simulink model "MMC_stack_centralized_HAAS_20260927"  (R2024b)
settings: Solver=FixedStepDiscrete  StartTime=t_init_sim  StopTime=sim_time  FixedStep=Ts  RelTol=1e-3
values from neighbouring files (symbols this model uses):
  a = 1    [script_MMC_stack_hackathon_NLM_centralized_HAAS_20260927.m]
  C1low1_active = 1    [script_MMC_stack_hackathon_NLM_centralized_HAAS_20260927.m]
  C2low1_active = 1    [script_MMC_stack_hackathon_NLM_centralized_HAAS_20260927.m]
  C_M_extra = C_m-twist_high_side_C    [script_MMC_stack_hackathon_NLM_centralized_HAAS_20260927.m]
  duty_cycle = 1.0    (= 1)    [script_MMC_stack_hackathon_NLM_centralized_HAAS_20260927.m]
  f0 = 50    [script_MMC_stack_hackathon_NLM_centralized_HAAS_20260927.m]
  feeder_current_lower_rate_limit = -10    [script_MMC_stack_hackathon_NLM_centralized_HAAS_20260927.m]    (also in twist_parameters.m = -500)
  feeder_current_tab = [0.328 0.217 0.162 0.132 0.109 0.094 0.083 0.075 0.068 0.062 0.058 0.054 ... (42 elements, 14x3)]    [feeder_current.mat]
  feeder_current_upper_rate_limit = 0.386/(20e-3)    (= 19.3)    [twist_parameters.m]
  is6VExternallySupplied = true    [script_MMC_stack_hackathon_NLM_centralized_HAAS_20260927.m]
  isFeederJumperOpen = true    [script_MMC_stack_hackathon_NLM_centralized_HAAS_20260927.m]
  L_arm = 30e-3    (= 0.03)    [script_MMC_stack_hackathon_NLM_centralized_HAAS_20260927.m]
  m = 1    [script_MMC_stack_hackathon_NLM_centralized_HAAS_20260927.m]
  N = 5    [script_MMC_stack_hackathon_NLM_centralized_HAAS_20260927.m]
  power_losses = false    [script_MMC_stack_hackathon_NLM_centralized_HAAS_20260927.m]
  R_p = R_s    (= 30)    [script_MMC_stack_hackathon_NLM_centralized_HAAS_20260927.m]
  R_s = 30    [script_MMC_stack_hackathon_NLM_centralized_HAAS_20260927.m]
  source_V = 0    [script_MMC_stack_hackathon_NLM_centralized_HAAS_20260927.m]
  Tcom_sample = round(Tcom / Ts)    [script_MMC_stack_hackathon_NLM_centralized_HAAS_20260927.m]
  time_charge = 0.1    [script_MMC_stack_hackathon_NLM_centralized_HAAS_20260927.m]
  time_decharge = 1.5    [script_MMC_stack_hackathon_NLM_centralized_HAAS_20260927.m]
  Ts = 1e-6    (= 1e-06)    [script_MMC_stack_hackathon_NLM_centralized_HAAS_20260927.m]
  twist_data_acquisition_delay = 50e-9    (= 5e-08)    [script_MMC_stack_hackathon_NLM_centralized_HAAS_20260927.m]    (also in twist_parameters.m)
  twist_data_sampling_period = 1/twist_freq_data_sampling    (= 5e-05)    [script_MMC_stack_hackathon_NLM_centralized_HAAS_20260927.m]    (also in twist_parameters.m)
  twist_dead_time = 200e-9    (= 2e-07)    [twist_parameters.m]
  twist_freq_switching = 200e3    (= 200000)    [twist_parameters.m]
  twist_high_side_adc_R = 1/(1/2e6 + 1/2e6 + 1/(330e3+5.6e3))    (= 251272.836178)    [twist_parameters.m]
  twist_high_side_C = 33e-6*4 + 4.7e-6*12    (= 0.0001884)    [twist_parameters.m]
  twist_high_side_feeder_R = 47e3+4.7e3    (= 51700)    [twist_parameters.m]
  twist_high_side_rC = 0.1    [twist_parameters.m]
  twist_low_side_adc_R = 150e3+470    (= 150470)    [twist_parameters.m]
  twist_low_side_C_ceramic = 3*4.7e-6    (= 1.41e-05)    [twist_parameters.m]
  twist_low_side_C_electrolytic = 47e-6    (= 4.7e-05)    [twist_parameters.m]
  twist_low_side_L = 33e-6    (= 3.3e-05)    [twist_parameters.m]
  twist_low_side_rC = 700e-3    (= 0.7)    [twist_parameters.m]
  twist_low_side_rL = 20e-3    (= 0.02)    [twist_parameters.m]
  twist_R_VCC = (tau_VCC/twist_high_side_C  - twist_high_side_rC)/(1-(tau_VCC/twist_high_side_C - twist_high_side_rC)/R_parallel)    (= 1110.74997822)    [twist_parameters.m]
  VDC = 48    [script_MMC_stack_hackathon_NLM_centralized_HAAS_20260927.m]
undefined symbols (not defined in the file or in its folder): C_SM, feeder_current, gcbh, R, sps_rtmsupport, twist_low_side_lC
libraries: spsSeriesRLCBranchLib x67, spsTriangleGeneratorLib x30, spsMosfetLib x30, spsCurrentMeasurementLib x21, spsVoltageMeasurementLib x17, spsControlledCurrentSourceLib x15, spsDiodeLib x11, spsIdealSwitchLib x10, spsControlledVoltageSourceLib x1, spsGroundLib x1, spspowerguiLib x1
(part 1 of 11)
settings Model: Creator=ana  LastModifiedBy=ana

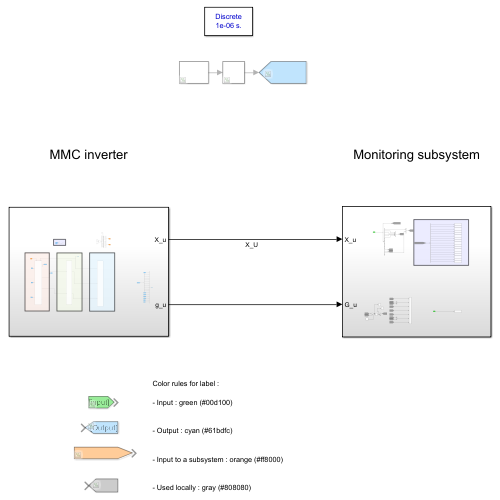
[thumbnail: Simulink's stored preview of the top-level diagram]
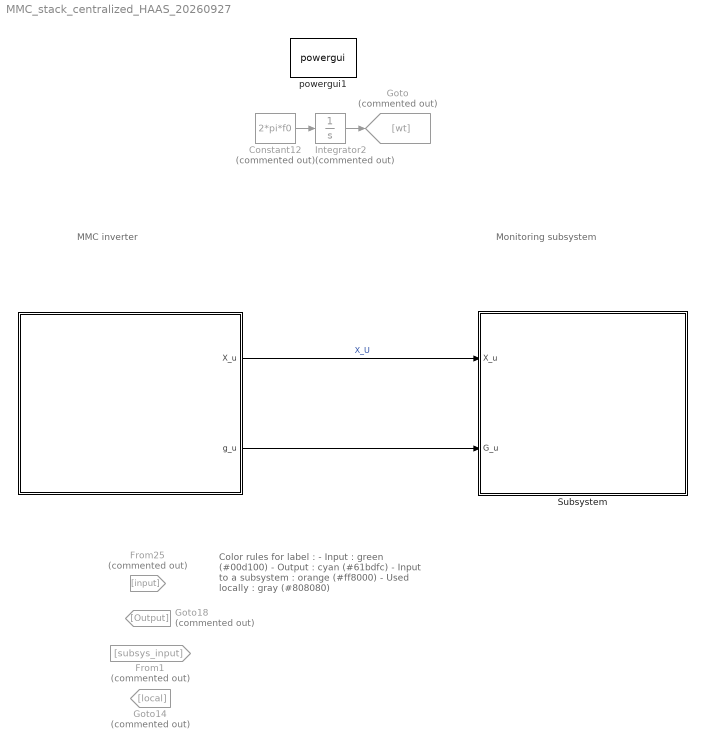
== system MMC_stack_centralized_HAAS_20260927 ==
  note: Color rules for label :
      |
      | - Input : green (#00d100)
      |
      |
      | - Output : cyan (#61bdfc)
      |
      |
      | - Input to a subsystem : orange (#ff8000)
      |
      |
      | - Used locally : gray (#808080)
  note: MMC inverter
  note: Monitoring subsystem
  " " : Subsystem
  Constant12 : Constant  Commented=on  Value=2*pi*f0
  From1 : From  Commented=on  GotoTag=subsys_input
  From25 : From  Commented=on  GotoTag=input
  Goto : Goto  Commented=on  GotoTag=wt
  Goto14 : Goto  Commented=on  GotoTag=local
  Goto18 : Goto  Commented=on  GotoTag=Output
  Integrator2 : Integrator  Commented=on
  Subsystem : Subsystem
  powergui1 : spspowerguiLib/powergui  Priority=1  SimulationMode=Discrete  SampleTime=Ts  frequency=60  Iterations=50  frequencyindice=0  Pbase=100e6  ErrMax=1e-4  UnitsV=V  UnitsW=W  buscounter=0  FunctionMessages=off  echomessages=off  EnableUseOfTLC=off  CurrentSourceSwitches=off  DisableSnubberDevices=off  DisableRonSwitches=off  DisableVfSwitches=off  DisplayEquations=off  AutomaticDiscreteSolvers=off  SolverType=Backward Euler  Interpol=off  ExternalGateDelay=off  methode=off  Ts=0  x0status=blocks  SPID=off  SwTol=0  HookPort=off  NonlinearTolerance=1e-4  nMaxIteration=100  ContinueOnMaxIteration=off  RestoreLinks=warning  ResistiveCurrentMeasurement=off  Frange=[0:2:500]  Ylog=off  Xlog=on  ShowGrid=off  save=off  variable=ZData  structure=0  ZoomFFT=off  StartTime=0.0  cycles=1  DisplayStyle=1  fundamental=60  FreqAxis=off  MaxFrequency=1000  frequencyindicesteady=1  RmsSteady=1  display=off
  wires:
  Constant12/1 -> Integrator2/1
  Integrator2/1 -> Goto/1
  " "/1(X_u) -> Subsystem/1(X_u)  "X_U"
  " "/2(g_u) -> Subsystem/2(G_u)

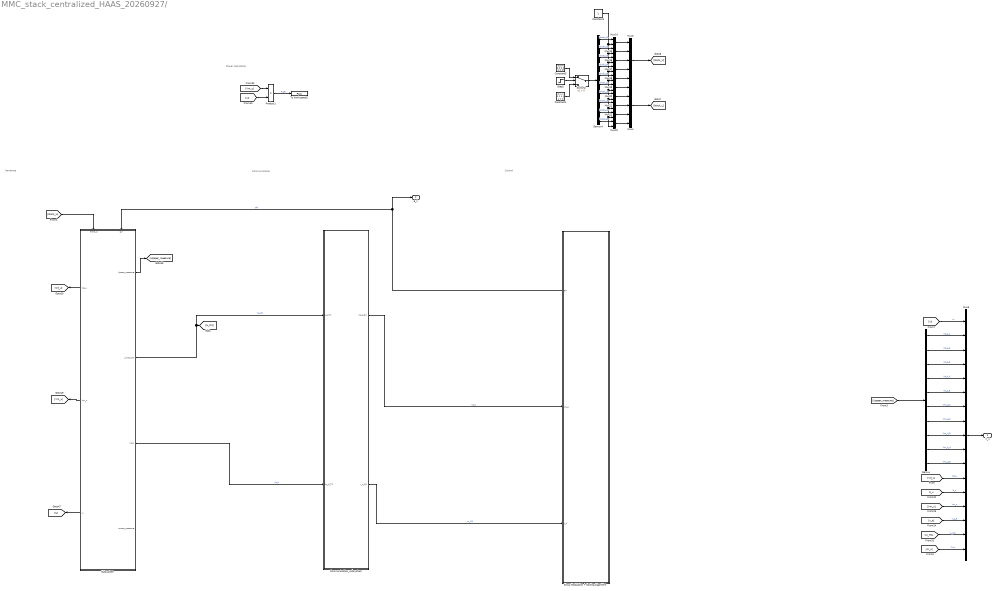
== system MMC_stack_centralized_HAAS_20260927/  ==
  note: Hardware
  note: Communication
  note: Power calculation
  note: Control
  Communication_subsystem : Subsystem
  Constant1 : Constant  Value=[1 1 1 1 1 1 1 1 1 1]
  Constant4 : Constant
  Constant5 : Constant  Value=[0 0 0 0 0 0 0 0 0 0]
  Demux : Demux  Outputs=10
  Demux4 : Demux  Outputs=10
  Mux{14..23} (10 alike) : Mux  Inputs=2
  Mux3 : Mux  Inputs=5
  Mux4 : Mux  Inputs=5
  Mux6 : Mux  Inputs=17
  Product1 : Product
  Sinus Modulation + Sorting Algorithm : Subsystem
      settings: PortSchema="{\"entries\":[{\"content\":{\"sides\":[{\"content\":{\"connectorIds\":[\"Out1\",\"In1\",\"In2\"]},\"type\":\"ConnectorPlacement.EquallySpacedRectSide\",\"uuid\":\"ad0c70b8-bd3d-4dd9-a5c4-c9fd50c7c997\"},{\"content\":{\"side\":\"RIGHT\"},\"type\":\"ConnectorPlacement.EquallySpacedRectSide\",\"uuid\":\"9cc59a2e-07a9-40e0-b04f-27b582e27098\"},{\"content\":{\"side\":\"TOP\"},\"type\":\"ConnectorPlacement.EquallySpacedRectSide\",\"uuid\":\"c85123d6-aff8-40c6-b6df-c7fa366f0af5\"}]},\"type\":\"ConnectorPlacement.EquallySpacedConnector\",\"uuid\":\"b1891b87-83b0-4249-9289-dc35b8395afb\"}],\"packageUris\":[\"http://schema.mathworks.com/mf0/Connector/R2020b\"],\"version\":\"1.0\"}"
  Step2 : Step  Time=time_charge  SampleTime=Ts
  Subsystem : Subsystem
      settings: PortSchema="{\"entries\":[{\"content\":{\"sides\":[{\"content\":{\"connectorIds\":[\"Out5\",\"Out6\",\"Out7\"]},\"type\":\"ConnectorPlacement.EquallySpacedRectSide\",\"uuid\":\"46d0b6b2-241e-4eaa-b5f4-7cb03ad6e4f0\"},{\"content\":{\"connectorIds\":[\"Out1\",\"Out2\",\"Out3\",\"Out4\"],\"side\":\"RIGHT\"},\"type\":\"ConnectorPlacement.EquallySpacedRectSide\",\"uuid\":\"f0391c40-5bbd-42ea-8549-0acba96c1793\"},{\"content\":{\"connectorIds\":[\"In1\",\"In2\"],\"side\":\"TOP\"},\"type\":\"ConnectorPlacement.EquallySpacedRectSide\",\"uuid\":\"1ede63b4-6869-46b3-8b67-84e7db18bcff\"},{\"content\":{\"side\":\"BOTTOM\"},\"type\":\"ConnectorPlacement.EquallySpacedRectSide\",\"uuid\":\"c0e3b199-6126-45b0-9783-8fc4162e2280\"}]},\"type\":\"ConnectorPlacement.EquallySpacedConnector\",\"uuid\":\"8bedc799-aa9e-49e4-9c41-8dbcca404e51\"}],\"packageUris\":[\"http://schema.mathworks.com/mf0/Connector/R2020b\"],\"version\":\"1.0\"}"
  Switch2 : Switch  Criteria=u2 > Threshold  SaturateOnIntegerOverflow=off  InputSameDT=off
  To Workspace2 : ToWorkspace  VariableName=Pout  SaveFormat=Structure With Time  SampleTime=-1
  X_u : Outport
  g_u : Outport  Port=2
  wires:
  Mux6/1 -> X_u/1
  Sinus Modulation + Sorting Algorithm/1(gU) -> Subsystem/2(gU), g_u/1  "gU"
  Communication_subsystem/2(I_U_RX) -> Sinus Modulation + Sorting Algorithm/2(I_U)  "Iu_M1"
  Product1/1 -> To Workspace2/1  "P_sa"
  [iu] -> Product1/2
  [iu] -> Mux6/1  "Iu"
  [Vd_u] -> Mux6/12  "Vd_u"
  [N_u] -> Mux6/13  "N_u"
  [Vm_u] -> Mux6/14  "Vm_u"
  [v_a] -> Mux6/15  "V_s_a"
  [iu_M1] -> Mux6/16  "Iu_M1"
  [Vm_u] -> Product1/1
  Communication_subsystem/1(Vc_U_RX) -> Sinus Modulation + Sorting Algorithm/1(Vc_U)  "Vc_U"
  [Uppper_measure] -> Demux/1
  Demux/1 -> Mux6/2  "Vc_U_1"
  Demux/2 -> Mux6/3  "Vc_U_2"
  Demux/3 -> Mux6/4  "Vc_U_3"
  Demux/4 -> Mux6/5  "Vc_U_4"
  Demux/5 -> Mux6/6  "Vc_U_5"
  Demux/6 -> Mux6/7  "Vm_U_1"
  Demux/7 -> Mux6/8  "Vm_U_2"
  Demux/8 -> Mux6/9  "Vm_U_3"
  Demux/9 -> Mux6/10  "Vm_U_4"
  Demux/10 -> Mux6/11  "Vm_U_5"
  [m_u] -> Mux6/17  "m_u"
  Subsystem/2(i_mod_M1) -> Communication_subsystem/1(I_U_TX), [iu_M1]  "IU_M1"
  Subsystem/3(Vc_U) -> Communication_subsystem/2(Vc_U_TX)  "Vc_U"
  Subsystem/7(iu) -> [iu]
  Subsystem/6(Vm_u) -> [Vm_u]
  Subsystem/5(Vd_u) -> [Vd_u]
  Subsystem/1(Upper_measure) -> [Uppper_measure]
  [block_U] -> Subsystem/1(block_U)
  Demux4/9 -> Mux22/1  "block_L4"
  Mux17/1 -> Mux3/4
  Mux22/1 -> Mux4/4
  Mux14/1 -> Mux3/1
  Demux4/1 -> Mux14/1  "block_U1"
  Constant5/1 -> Switch2/1
  Demux4/3 -> Mux16/1  "block_U3"
  Mux21/1 -> Mux4/3
  Switch2/1 -> Demux4/1
  Demux4/5 -> Mux18/1  "block_U5"
  Demux4/10 -> Mux23/1  "block_L5"
  Constant1/1 -> Switch2/3
  Demux4/7 -> Mux20/1  "block_L2"
  Mux19/1 -> Mux4/1
  Mux23/1 -> Mux4/5
  Demux4/2 -> Mux15/1  "block_U2"
  Constant4/1 -> Mux23/2, Mux22/2, Mux21/2, Mux20/2, Mux19/2, Mux18/2, Mux17/2, Mux16/2, Mux15/2, Mux14/2
  Demux4/6 -> Mux19/1  "block_L1"
  Demux4/8 -> Mux21/1  "block_L3"
  Mux16/1 -> Mux3/3
  Mux15/1 -> Mux3/2
  Mux20/1 -> Mux4/2
  Mux18/1 -> Mux3/5
  Demux4/4 -> Mux17/1  "block_U4"
  Step2/1 -> Switch2/2
  Mux3/1 -> [block_U]
  Mux4/1 -> [block_L]

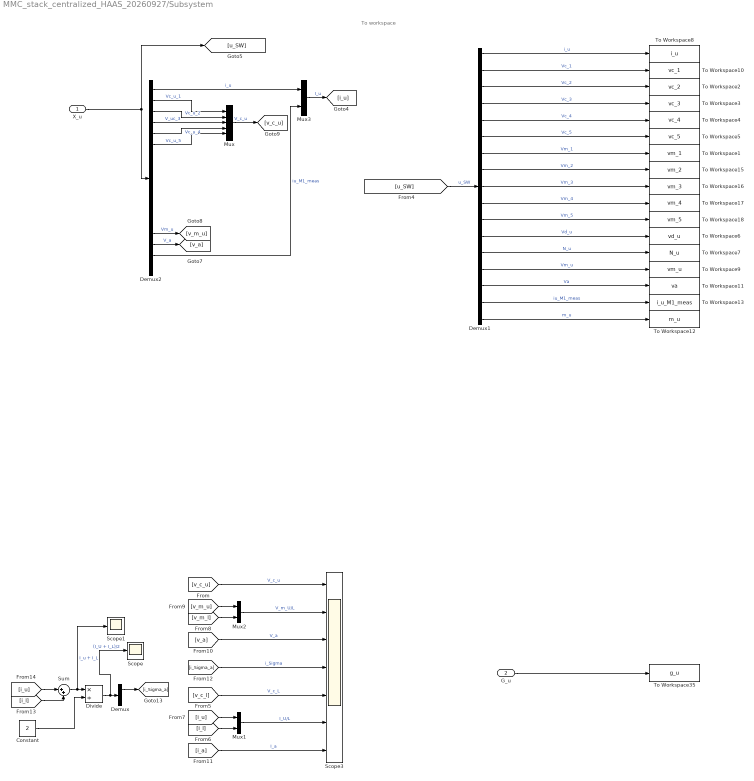
== system MMC_stack_centralized_HAAS_20260927/Subsystem ==
  note: To workspace
  X_u : Inport
  G_u : Inport  Port=2
  Constant : Constant  Value=2
  Demux : Demux  Outputs=2
  Demux1 : Demux  Outputs=17
  Demux2 : Demux  Outputs=17
  Divide : Product  Inputs=*/
  Mux : Mux  Inputs=5
  Mux1 : Mux  Inputs=2
  Mux2 : Mux  Inputs=2
  Mux3 : Mux  Inputs=2
  Scope : Scope
  Scope1 : Scope
  Scope3 : Scope  NumInputPorts=7
  Sum : Sum  Inputs=|++
  To Workspace1 : ToWorkspace  VariableName=vm_1  SaveFormat=Structure With Time  SampleTime=-1
  To Workspace10 : ToWorkspace  VariableName=vc_1  SaveFormat=Structure With Time  SampleTime=-1
  To Workspace11 : ToWorkspace  VariableName=va  SaveFormat=Structure With Time  SampleTime=-1
  To Workspace12 : ToWorkspace  VariableName=m_u  SaveFormat=Structure With Time  SampleTime=-1
  To Workspace13 : ToWorkspace  VariableName=i_u_M1_meas  SaveFormat=Structure With Time  SampleTime=-1
  To Workspace15 : ToWorkspace  VariableName=vm_2  SaveFormat=Structure With Time  SampleTime=-1
  To Workspace16 : ToWorkspace  VariableName=vm_3  SaveFormat=Structure With Time  SampleTime=-1
  To Workspace17 : ToWorkspace  VariableName=vm_4  SaveFormat=Structure With Time  SampleTime=-1
  To Workspace18 : ToWorkspace  VariableName=vm_5  SaveFormat=Structure With Time  SampleTime=-1
  To Workspace2 : ToWorkspace  VariableName=vc_2  SaveFormat=Structure With Time  SampleTime=-1
  To Workspace3 : ToWorkspace  VariableName=vc_3  SaveFormat=Structure With Time  SampleTime=-1
  To Workspace35 : ToWorkspace  VariableName=g_u  SaveFormat=Structure With Time  SampleTime=-1
  To Workspace4 : ToWorkspace  VariableName=vc_4  SaveFormat=Structure With Time  SampleTime=-1
  To Workspace5 : ToWorkspace  VariableName=vc_5  SaveFormat=Structure With Time  SampleTime=-1
  To Workspace6 : ToWorkspace  VariableName=vd_u  SaveFormat=Structure With Time  SampleTime=-1
  To Workspace7 : ToWorkspace  VariableName=N_u  SaveFormat=Structure With Time  SampleTime=-1
  To Workspace8 : ToWorkspace  VariableName=i_u  SaveFormat=Structure With Time  SampleTime=-1
  To Workspace9 : ToWorkspace  VariableName=vm_u  SaveFormat=Structure With Time  SampleTime=-1
  wires:
  Demux1/4 -> To Workspace3/1  "Vc_3"
  Demux2/14 -> [v_m_u]  "Vm_u"
  Demux1/2 -> To Workspace10/1  "Vc_1"
  Demux1/14 -> To Workspace9/1  "Vm_u"
  Mux2/1 -> Scope3/2  "V_m_U/L"
  Demux1/7 -> To Workspace1/1  "Vm_1"
  Demux2/1 -> Mux3/1  "i_u"
  Demux2/4 -> Mux/3  "V_uc_3"
  [v_m_u] -> Mux2/1
  [i_a] -> Scope3/7  "I_a"
  X_u/1 -> Demux2/1, [u_SW]
  Demux2/15 -> [v_a]  "V_a"
  Demux2/16 -> Mux3/2  "iu_M1_meas"
  [i_l] -> Sum/2
  Demux1/11 -> To Workspace18/1  "Vm_5"
  Demux1/13 -> To Workspace7/1  "N_u"
  Demux2/3 -> Mux/2  "Vc_u_2"
  [i_u] -> Mux1/1
  Demux1/5 -> To Workspace4/1  "Vc_4"
  Mux3/1 -> [i_u]  "I_u"
  Constant/1 -> Divide/2
  Sum/1 -> Scope1/1, Divide/1  "I_u + I_L"
  Divide/1 -> Scope/1, Demux/1  "(I_U + I_L)/2"
  Demux1/3 -> To Workspace2/1  "Vc_2"
  Demux1/16 -> To Workspace13/1  "iu_M1_meas"
  Demux2/5 -> Mux/4  "Vc_u_4"
  [v_a] -> Scope3/3  "V_a"
  Demux1/10 -> To Workspace17/1  "Vm_4"
  [i_l] -> Mux1/2
  [u_SW] -> Demux1/1  "u_SW"
  Demux1/17 -> To Workspace12/1  "m_u"
  Demux1/15 -> To Workspace11/1  "Va"
  Demux1/12 -> To Workspace6/1  "Vd_u"
  Demux2/2 -> Mux/1  "Vc_u_1"
  Demux1/9 -> To Workspace16/1  "Vm_3"
  Demux/1 -> [i_Sigma_a]
  [v_c_l] -> Scope3/5  "V_c_L"
  Demux2/6 -> Mux/5  "Vc_u_5"
  Demux1/8 -> To Workspace15/1  "Vm_2"
  [v_c_u] -> Scope3/1  "V_c_u"
  Demux1/6 -> To Workspace5/1  "Vc_5"
  Demux1/1 -> To Workspace8/1  "i_u"
  [v_m_l] -> Mux2/2
  [i_u] -> Sum/1
  [i_Sigma_a] -> Scope3/4  "i_Sigma"
  Mux1/1 -> Scope3/6  "I_U/L"
  Mux/1 -> [v_c_u]  "V_c_u"
  G_u/1 -> To Workspace35/1

== system MMC_stack_centralized_HAAS_20260927/ /Communication_subsystem ==
  I_U_TX : Inport
  Vc_U_TX : Inport  Port=2
  Communication architecture : Subsystem
      settings: PortSchema="{\"entries\":[{\"content\":{\"sides\":[{\"content\":{\"connectorIds\":[\"In1\",\"In2\",\"Out2\",\"In3\",\"Out3\",\"In4\",\"Out4\",\"In5\",\"Out5\",\"Out6\"]},\"type\":\"ConnectorPlacement.EquallySpacedRectSide\",\"uuid\":\"574f1c32-5c90-4713-aad2-348eca17c1e3\"},{\"content\":{\"connectorIds\":[\"Out1\"],\"side\":\"RIGHT\"},\"type\":\"ConnectorPlacement.EquallySpacedRectSide\",\"uuid\":\"f8c779b5-ecb7-4a42-bc9c-e4bb2f97a0b3\"},{\"content\":{\"side\":\"TOP\"},\"type\":\"ConnectorPlacement.EquallySpacedRectSide\",\"uuid\":\"aac8d141-a504-4135-a079-04baa73dba14\"}]},\"type\":\"ConnectorPlacement.EquallySpacedConnector\",\"uuid\":\"cbc34fff-d47b-42f9-bfde-18f06952df39\"}],\"packageUris\":[\"http://schema.mathworks.com/mf0/Connector/R2020b\"],\"version\":\"1.0\"}"
  Demux2 : Demux  Outputs=12
  Mux : Mux  Inputs=2
  Scope : Scope
  Sync : DiscretePulseGenerator  Period=round((200e-6)/Ts)  PulseWidth=round(20e-6/Ts)  SampleTime=Ts
  Term_RX_{7..12} (6 alike) : Terminator
  Upper_arm : Subsystem
      settings: PortSchema="{\"entries\":[{\"content\":{\"sides\":[{\"content\":{\"connectorIds\":[\"In1\",\"In2\"]},\"type\":\"ConnectorPlacement.EquallySpacedRectSide\",\"uuid\":\"e2448297-5920-4ed4-b9a5-463387ed0389\"},{\"content\":{\"connectorIds\":[\"Out1\",\"In3\",\"Out2\",\"In4\",\"Out3\",\"In5\",\"Out4\",\"In6\",\"Out5\",\"In7\"],\"side\":\"RIGHT\"},\"type\":\"ConnectorPlacement.EquallySpacedRectSide\",\"uuid\":\"29ac6558-0bf6-4432-86a8-2cc792ef1820\"},{\"content\":{\"connectorIds\":[\"Out6\"],\"side\":\"TOP\"},\"type\":\"ConnectorPlacement.EquallySpacedRectSide\",\"uuid\":\"fe3a666d-35d9-4a5d-8998-edcd1cd24e1f\"}]},\"type\":\"ConnectorPlacement.EquallySpacedConnector\",\"uuid\":\"a9564cd0-ea30-4b39-994d-f524846fcfc7\"}],\"packageUris\":[\"http://schema.mathworks.com/mf0/Connector/R2020b\"],\"version\":\"1.0\"}"
  Vector Concatenate : Concatenate  NumInputs=5
  Vc_U_RX : Outport
  I_U_RX : Outport  Port=2
  wires:
  Vc_U_TX/1 -> Mux/1
  Mux/1 -> Upper_arm/1(upper_arm_info)
  Upper_arm/1(M1_TX_signal) -> Communication architecture/1(M1_TX_Signal)
  Upper_arm/2(M2_TX_signal) -> Communication architecture/2(M2_TX_Signal)
  Upper_arm/3(M3_TX_signal) -> Communication architecture/3(M3_TX_Signal)
  Upper_arm/4(M4_TX_signal) -> Communication architecture/4(M4_TX_Signal)
  Upper_arm/5(M5_TX_signal) -> Communication architecture/5(M5_TX_Signal)
  I_U_TX/1 -> Mux/2
  Sync/1 -> Upper_arm/2(sync)
  Upper_arm/6(RX_Variables) -> [RX_variable]
  [RX_variable] -> Demux2/1
  Demux2/1 -> Scope/1, Vector Concatenate/1  "Vc_u_1"
  Demux2/2 -> Vector Concatenate/2  "Vc_u_2"
  Demux2/3 -> Vector Concatenate/3  "Vc_u_3"
  Demux2/4 -> Vector Concatenate/4  "Vc_u_4"
  Demux2/5 -> Vector Concatenate/5  "Vc_u_5"
  Vector Concatenate/1 -> Vc_U_RX/1
  Demux2/6 -> I_U_RX/1
  Communication architecture/2(M2_RX_Signal) -> Upper_arm/4(M2_RX_signal)
  Communication architecture/3(M3_RX_Signal) -> Upper_arm/5(M3_RX_signal)
  Communication architecture/4(M4_RX_Signal) -> Upper_arm/6(M4_RX_signal)
  Communication architecture/5(M5_RX_Signal) -> Upper_arm/7(M5_RX_signal)
  Communication architecture/6(M1_RX_Signal) -> Upper_arm/3(M1_RX_signal)
  Demux2/7 -> Term_RX_7/1
  Demux2/8 -> Term_RX_8/1
  Demux2/9 -> Term_RX_9/1
  Demux2/10 -> Term_RX_10/1
  Demux2/11 -> Term_RX_11/1
  Demux2/12 -> Term_RX_12/1

== system MMC_stack_centralized_HAAS_20260927/ /Sinus Modulation + Sorting Algorithm ==
  note: Sorting and CVB algorithm - Upper and Lower stacks
  note: Gate assignement - Modules MCUs
  Vc_U : Inport
  I_U : Inport  Port=2
  Constant5 : Constant
  Constant6 : Constant  Value=2
  Constant7 : Constant  Value=3
  Constant8 : Constant  Value=4
  Constant9 : Constant  Value=5
  M1 MCU : Subsystem
  M2 MCU : Subsystem
  M3 MCU : Subsystem
  M4 MCU : Subsystem
  M5 MCU : Subsystem
  Mux : Mux  Inputs=5
  Supervisor MCU : Subsystem
  gU : Outport
  tag scope: g_u_supervisor=global
  wires:
  M1 MCU/1(g_unitaire_stack) -> Mux/1
  M2 MCU/1(g_unitaire_stack) -> Mux/2
  M3 MCU/1(g_unitaire_stack) -> Mux/3
  M4 MCU/1(g_unitaire_stack) -> Mux/4
  M5 MCU/1(g_unitaire_stack) -> Mux/5
  Constant5/1 -> M1 MCU/2(M_number)
  Constant6/1 -> M2 MCU/2(M_number)
  Constant7/1 -> M3 MCU/2(M_number)
  Constant8/1 -> M4 MCU/2(M_number)
  Constant9/1 -> M5 MCU/2(M_number)
  I_U/1 -> Supervisor MCU/2(I_U)
  Vc_U/1 -> Supervisor MCU/1(Vc_U)
  Supervisor MCU/1(gU) -> [g_u_supervisor]
  [g_u_supervisor] -> M5 MCU/1(g_u), M4 MCU/1(g_u), M3 MCU/1(g_u), M2 MCU/1(g_u), M1 MCU/1(g_u)
  Mux/1 -> gU/1

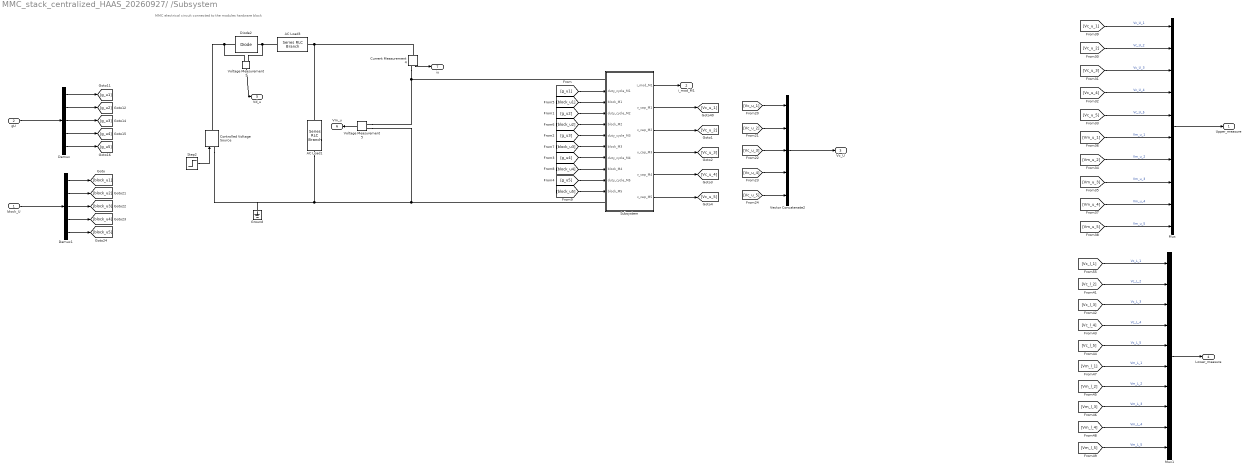
== system MMC_stack_centralized_HAAS_20260927/ /Subsystem ==
  note: MMC electrical circuit connected to the modules hardware block
  block_U : Inport
  gU : Inport  Port=2
  AC Load1 : spsSeriesRLCBranchLib/Series RLC Branch  LConnTagsString=__new0  RConnTagsString=__new0  BranchType=R  Resistance=R_p  Inductance=L_arm  SetiL0=off  InitialCurrent=0  Capacitance=C_SM  Setx0=off  InitialVoltage=0  Measurements=None
  AC Load3 : spsSeriesRLCBranchLib/Series RLC Branch  LConnTagsString=__new0  RConnTagsString=__new0  BranchType=R  Resistance=R_s  Inductance=L_arm  SetiL0=off  InitialCurrent=0  Capacitance=C_SM  Setx0=off  InitialVoltage=0  Measurements=None
  Controlled Voltage Source : spsControlledVoltageSourceLib/Controlled Voltage Source  Initialize=on  Source_Type=DC  Amplitude=0  Phase=0  Frequency=0  Measurements=None
  Current Measurement4 : spsCurrentMeasurementLib/Current Measurement  PhasorSimulation=off  OutputType=Complex  PSBequivalent=0
  Demux : Demux  Outputs=5
  Demux1 : Demux  Outputs=5
  Diode2 : spsDiodeLib/Diode  Ron=0.001  Lon=0  Vf=0.8  IC=0  UseSnubber=0  Rs=1e5  Cs=inf  Measurements=off
  Ground : spsGroundLib/Ground  LConnTagsString=a
  Mux : Mux  Inputs=10
  Mux1 : Mux  Inputs=10
  Step2 : Step  Time=time_decharge  Before=VDC  After=0  SampleTime=0
  Subsystem : Subsystem
      settings: PortSchema="{\"entries\":[{\"content\":{\"sides\":[{\"content\":{\"connectorIds\":[\"LConn1\",\"In1\",\"In2\",\"In3\",\"In4\",\"In5\",\"In6\",\"In7\",\"In8\",\"In9\",\"In10\",\"LConn2\"]},\"type\":\"ConnectorPlacement.EquallySpacedRectSide\",\"uuid\":\"af96ca56-9fdb-47ea-8e31-50f481daafc4\"},{\"content\":{\"connectorIds\":[\"Out1\",\"Out2\",\"Out3\",\"Out4\",\"Out5\",\"Out6\"],\"side\":\"RIGHT\"},\"type\":\"ConnectorPlacement.EquallySpacedRectSide\",\"uuid\":\"66f6256f-049a-4c8a-aad5-8d93b148b037\"},{\"content\":{\"side\":\"TOP\"},\"type\":\"ConnectorPlacement.EquallySpacedRectSide\",\"uuid\":\"596eb3e1-7761-4783-802e-d9df31b3a9c1\"}]},\"type\":\"ConnectorPlacement.EquallySpacedConnector\",\"uuid\":\"34c6ade5-a2f4-48d8-9a9b-6856a5a88d76\"}],\"packageUris\":[\"http://schema.mathworks.com/mf0/Connector/R2020b\"],\"version\":\"1.0\"}"
  Vector Concatenate2 : Concatenate  NumInputs=5
  Voltage Measurement5 : spsVoltageMeasurementLib/Voltage Measurement  PhasorSimulation=off  OutputType=Complex  PSBequivalent=0
  Voltage Measurement7 : spsVoltageMeasurementLib/Voltage Measurement  PhasorSimulation=off  OutputType=Complex  PSBequivalent=0
  Upper_measure : Outport
  i_mod_M1 : Outport  Port=2
  Vc_U : Outport  Port=3
  Lower_measure : Outport  Port=4
  Vd_u : Outport  Port=5
  Vm_u : Outport  Port=6
  iu : Outport  Port=7
  wires:
  Voltage Measurement7/1 -> Vd_u/1
  Step2/1 -> Controlled Voltage Source/1
  Voltage Measurement5/1 -> Vm_u/1
  [g_u1] -> Subsystem/1(duty_cycle_M1)
  [block_u1] -> Subsystem/2(block_M1)
  [g_u2] -> Subsystem/3(duty_cycle_M2)
  [block_u2] -> Subsystem/4(block_M2)
  [g_u3] -> Subsystem/5(duty_cycle_M3)
  [block_u3] -> Subsystem/6(block_M3)
  [g_u4] -> Subsystem/7(duty_cycle_M4)
  [block_u4] -> Subsystem/8(block_M4)
  [g_u5] -> Subsystem/9(duty_cycle_M5)
  [block_u5] -> Subsystem/10(block_M5)
  Subsystem/1(i_mod_M1) -> i_mod_M1/1
  Subsystem/6(v_cap_M5) -> [Vc_u_5]
  Subsystem/5(v_cap_M4) -> [Vc_u_4]
  Subsystem/2(v_cap_M1) -> [Vc_u_1]
  Subsystem/3(v_cap_M2) -> [Vc_u_2]
  Subsystem/4(v_cap_M3) -> [Vc_u_3]
  Current Measurement4/1 -> iu/1
  Vector Concatenate2/1 -> Vc_U/1
  Demux/2 -> [g_u2]
  Demux/5 -> [g_u5]
  Demux1/5 -> [block_u5]
  Demux/4 -> [g_u4]
  Demux/3 -> [g_u3]
  Demux1/1 -> [block_u1]
  gU/1 -> Demux/1
  block_U/1 -> Demux1/1
  Demux1/2 -> [block_u2]
  Demux/1 -> [g_u1]
  Demux1/4 -> [block_u4]
  Demux1/3 -> [block_u3]
  [Vc_u_1] -> Vector Concatenate2/1
  [Vc_u_2] -> Vector Concatenate2/2
  [Vc_u_3] -> Vector Concatenate2/3
  [Vc_u_4] -> Vector Concatenate2/4
  [Vc_u_5] -> Vector Concatenate2/5
  [Vc_u_1] -> Mux/1  "Vc_U_1"
  [Vm_u_5] -> Mux/10  "Vm_u_5"
  [Vm_u_4] -> Mux/9  "Vm_u_4"
  [Vc_u_3] -> Mux/3  "Vc_U_3"
  [Vm_u_3] -> Mux/8  "Vm_u_3"
  [Vc_u_2] -> Mux/2  "Vc_U_2"
  [Vm_u_2] -> Mux/7  "Vm_u_2"
  [Vm_u_1] -> Mux/6  "Vm_u_1"
  [Vc_u_4] -> Mux/4  "Vc_U_4"
  [Vc_u_5] -> Mux/5  "Vc_U_5"
  [Vc_l_2] -> Mux1/2  "Vc_L_2"
  [Vm_l_2] -> Mux1/7  "Vm_L_2"
  [Vc_l_1] -> Mux1/1  "Vc_L_1"
  [Vm_l_4] -> Mux1/9  "Vm_L_4"
  [Vm_l_5] -> Mux1/10  "Vm_L_5"
  [Vm_l_1] -> Mux1/6  "Vm_L_1"
  [Vm_l_3] -> Mux1/8  "Vm_L_3"
  [Vc_l_3] -> Mux1/3  "Vc_L_3"
  [Vc_l_5] -> Mux1/5  "Vc_L_5"
  [Vc_l_4] -> Mux1/4  "Vc_L_4"
  Mux1/1 -> Lower_measure/1
  Mux/1 -> Upper_measure/1
  connections:
  Diode2/RConn1 -- AC Load3/LConn1 -- Voltage Measurement7/LConn2
  Current Measurement4/RConn1 -- Voltage Measurement5/LConn1 -- Subsystem/LConn1
  Voltage Measurement5/LConn2 -- Controlled Voltage Source/LConn1 -- Ground/LConn1 -- AC Load1/RConn1 -- Subsystem/LConn2
  Voltage Measurement7/LConn1 -- Controlled Voltage Source/RConn1 -- Diode2/LConn1
  AC Load1/LConn1 -- Current Measurement4/LConn1 -- AC Load3/RConn1

== system MMC_stack_centralized_HAAS_20260927/ /Communication_subsystem/Communication architecture ==
  M1_TX_Signal : Inport
  M2_TX_Signal : Inport  Port=2
  M3_TX_Signal : Inport  Port=3
  M4_TX_Signal : Inport  Port=4
  M5_TX_Signal : Inport  Port=5
  MATLAB Function : MATLAB Function  Commented=on  TreatAsAtomicUnit=on
  RX_Signal : Outport
  M2_RX_Signal : Outport  Port=2
  M3_RX_Signal : Outport  Port=3
  M4_RX_Signal : Outport  Port=4
  M5_RX_Signal : Outport  Port=5
  M1_RX_Signal : Outport  Port=6
  wires:
  MATLAB Function/1(bus_signal) -> RX_Signal/1
  M4_TX_Signal/1 -> M5_RX_Signal/1
  M5_TX_Signal/1 -> M1_RX_Signal/1
  M1_TX_Signal/1 -> M2_RX_Signal/1
  M2_TX_Signal/1 -> M3_RX_Signal/1
  M3_TX_Signal/1 -> M4_RX_Signal/1

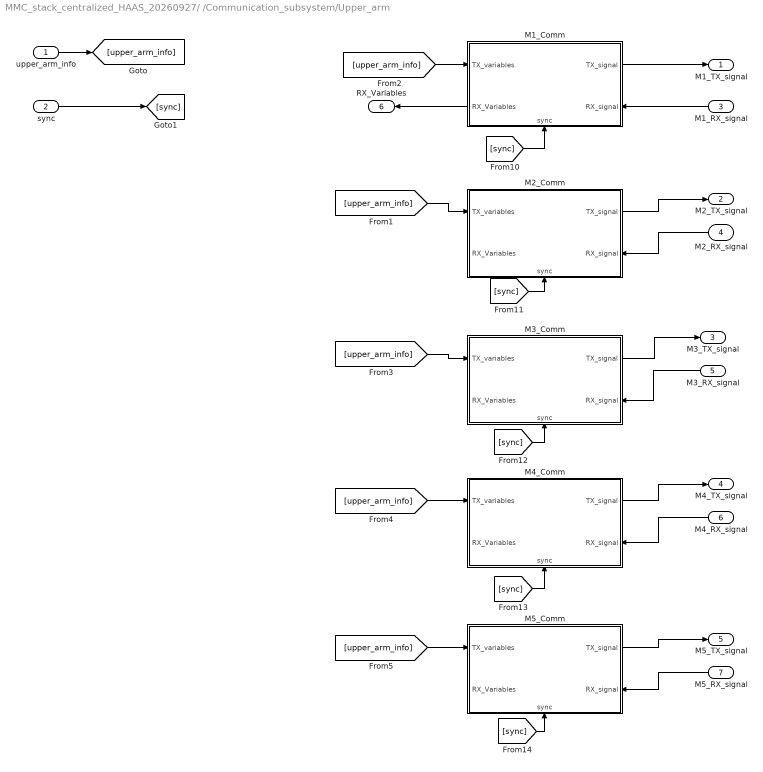
== system MMC_stack_centralized_HAAS_20260927/ /Communication_subsystem/Upper_arm ==
  upper_arm_info : Inport
  sync : Inport  Port=2
  M1_RX_signal : Inport  Port=3
  M2_RX_signal : Inport  Port=4
  M3_RX_signal : Inport  Port=5
  M4_RX_signal : Inport  Port=6
  M5_RX_signal : Inport  Port=7
  M1_Comm : Subsystem
      settings: PortSchema="{\"entries\":[{\"content\":{\"sides\":[{\"content\":{\"connectorIds\":[\"In1\",\"Out2\"]},\"type\":\"ConnectorPlacement.EquallySpacedRectSide\",\"uuid\":\"c3733cfa-9814-4ae5-a55a-8e5b6f8a57d7\"},{\"content\":{\"connectorIds\":[\"Out1\",\"In3\"],\"side\":\"RIGHT\"},\"type\":\"ConnectorPlacement.EquallySpacedRectSide\",\"uuid\":\"d16535d3-81ee-4162-a646-15cef1f1639a\"},{\"content\":{\"side\":\"TOP\"},\"type\":\"ConnectorPlacement.EquallySpacedRectSide\",\"uuid\":\"672d53ef-99b6-4fa6-8351-42251f607454\"},{\"content\":{\"connectorIds\":[\"In2\"],\"side\":\"BOTTOM\"},\"type\":\"ConnectorPlacement.EquallySpacedRectSide\",\"uuid\":\"a9bd7512-44c2-4af9-8132-4c17be33b3c2\"}]},\"type\":\"ConnectorPlacement.EquallySpacedConnector\",\"uuid\":\"554aea8b-7fd0-4035-ac75-3acab423d605\"}],\"packageUris\":[\"http://schema.mathworks.com/mf0/Connector/R2020b\"],\"version\":\"1.0\"}"
  M2_Comm : Subsystem
      settings: PortSchema="{\"entries\":[{\"content\":{\"sides\":[{\"content\":{\"connectorIds\":[\"In1\",\"Out2\"]},\"type\":\"ConnectorPlacement.EquallySpacedRectSide\",\"uuid\":\"47077a1e-eba1-4129-8203-93262b2de465\"},{\"content\":{\"connectorIds\":[\"Out1\",\"In3\"],\"side\":\"RIGHT\"},\"type\":\"ConnectorPlacement.EquallySpacedRectSide\",\"uuid\":\"701fdbad-c928-45f3-8ba2-a14f680316f8\"},{\"content\":{\"side\":\"TOP\"},\"type\":\"ConnectorPlacement.EquallySpacedRectSide\",\"uuid\":\"d648951b-caea-4569-a411-8455254fdbc0\"},{\"content\":{\"connectorIds\":[\"In2\"],\"side\":\"BOTTOM\"},\"type\":\"ConnectorPlacement.EquallySpacedRectSide\",\"uuid\":\"d4b1d2d6-b4a1-4e2c-9ca6-248db102ef7c\"}]},\"type\":\"ConnectorPlacement.EquallySpacedConnector\",\"uuid\":\"7c33ff72-602e-419f-9c2d-5eefc0d60400\"}],\"packageUris\":[\"http://schema.mathworks.com/mf0/Connector/R2020b\"],\"version\":\"1.0\"}"
  M3_Comm : Subsystem
      settings: PortSchema="{\"entries\":[{\"content\":{\"sides\":[{\"content\":{\"connectorIds\":[\"In1\",\"Out2\"]},\"type\":\"ConnectorPlacement.EquallySpacedRectSide\",\"uuid\":\"47077a1e-eba1-4129-8203-93262b2de465\"},{\"content\":{\"connectorIds\":[\"Out1\",\"In3\"],\"side\":\"RIGHT\"},\"type\":\"ConnectorPlacement.EquallySpacedRectSide\",\"uuid\":\"701fdbad-c928-45f3-8ba2-a14f680316f8\"},{\"content\":{\"side\":\"TOP\"},\"type\":\"ConnectorPlacement.EquallySpacedRectSide\",\"uuid\":\"d648951b-caea-4569-a411-8455254fdbc0\"},{\"content\":{\"connectorIds\":[\"In2\"],\"side\":\"BOTTOM\"},\"type\":\"ConnectorPlacement.EquallySpacedRectSide\",\"uuid\":\"d4b1d2d6-b4a1-4e2c-9ca6-248db102ef7c\"}]},\"type\":\"ConnectorPlacement.EquallySpacedConnector\",\"uuid\":\"7c33ff72-602e-419f-9c2d-5eefc0d60400\"}],\"packageUris\":[\"http://schema.mathworks.com/mf0/Connector/R2020b\"],\"version\":\"1.0\"}"
  M4_Comm : Subsystem
      settings: PortSchema="{\"entries\":[{\"content\":{\"sides\":[{\"content\":{\"connectorIds\":[\"In1\",\"Out2\"]},\"type\":\"ConnectorPlacement.EquallySpacedRectSide\",\"uuid\":\"47077a1e-eba1-4129-8203-93262b2de465\"},{\"content\":{\"connectorIds\":[\"Out1\",\"In3\"],\"side\":\"RIGHT\"},\"type\":\"ConnectorPlacement.EquallySpacedRectSide\",\"uuid\":\"701fdbad-c928-45f3-8ba2-a14f680316f8\"},{\"content\":{\"side\":\"TOP\"},\"type\":\"ConnectorPlacement.EquallySpacedRectSide\",\"uuid\":\"d648951b-caea-4569-a411-8455254fdbc0\"},{\"content\":{\"connectorIds\":[\"In2\"],\"side\":\"BOTTOM\"},\"type\":\"ConnectorPlacement.EquallySpacedRectSide\",\"uuid\":\"d4b1d2d6-b4a1-4e2c-9ca6-248db102ef7c\"}]},\"type\":\"ConnectorPlacement.EquallySpacedConnector\",\"uuid\":\"7c33ff72-602e-419f-9c2d-5eefc0d60400\"}],\"packageUris\":[\"http://schema.mathworks.com/mf0/Connector/R2020b\"],\"version\":\"1.0\"}"
  M5_Comm : Subsystem
      settings: PortSchema="{\"entries\":[{\"content\":{\"sides\":[{\"content\":{\"connectorIds\":[\"In1\",\"Out2\"]},\"type\":\"ConnectorPlacement.EquallySpacedRectSide\",\"uuid\":\"47077a1e-eba1-4129-8203-93262b2de465\"},{\"content\":{\"connectorIds\":[\"Out1\",\"In3\"],\"side\":\"RIGHT\"},\"type\":\"ConnectorPlacement.EquallySpacedRectSide\",\"uuid\":\"701fdbad-c928-45f3-8ba2-a14f680316f8\"},{\"content\":{\"side\":\"TOP\"},\"type\":\"ConnectorPlacement.EquallySpacedRectSide\",\"uuid\":\"d648951b-caea-4569-a411-8455254fdbc0\"},{\"content\":{\"connectorIds\":[\"In2\"],\"side\":\"BOTTOM\"},\"type\":\"ConnectorPlacement.EquallySpacedRectSide\",\"uuid\":\"d4b1d2d6-b4a1-4e2c-9ca6-248db102ef7c\"}]},\"type\":\"ConnectorPlacement.EquallySpacedConnector\",\"uuid\":\"7c33ff72-602e-419f-9c2d-5eefc0d60400\"}],\"packageUris\":[\"http://schema.mathworks.com/mf0/Connector/R2020b\"],\"version\":\"1.0\"}"
  M1_TX_signal : Outport
  M2_TX_signal : Outport  Port=2
  M3_TX_signal : Outport  Port=3
  M4_TX_signal : Outport  Port=4
  M5_TX_signal : Outport  Port=5
  RX_Variables : Outport  Port=6
  wires:
  [upper_arm_info] -> M5_Comm/1(TX_variables)
  M4_Comm/1(TX_signal) -> M4_TX_signal/1
  [upper_arm_info] -> M1_Comm/1(TX_variables)
  [upper_arm_info] -> M4_Comm/1(TX_variables)
  M3_Comm/1(TX_signal) -> M3_TX_signal/1
  M2_Comm/1(TX_signal) -> M2_TX_signal/1
  [upper_arm_info] -> M2_Comm/1(TX_variables)
  [upper_arm_info] -> M3_Comm/1(TX_variables)
  M1_RX_signal/1 -> M1_Comm/3(RX_signal)
  [sync] -> M3_Comm/2(sync)
  M3_RX_signal/1 -> M3_Comm/3(RX_signal)
  [sync] -> M5_Comm/2(sync)
  [sync] -> M4_Comm/2(sync)
  [sync] -> M1_Comm/2(sync)
  M5_RX_signal/1 -> M5_Comm/3(RX_signal)
  M1_Comm/1(TX_signal) -> M1_TX_signal/1
  M2_RX_signal/1 -> M2_Comm/3(RX_signal)
  [sync] -> M2_Comm/2(sync)
  M5_Comm/1(TX_signal) -> M5_TX_signal/1
  M4_RX_signal/1 -> M4_Comm/3(RX_signal)
  upper_arm_info/1 -> [upper_arm_info]
  sync/1 -> [sync]
  M1_Comm/2(RX_Variables) -> RX_Variables/1

== system MMC_stack_centralized_HAAS_20260927/ /Sinus Modulation + Sorting Algorithm/M1 MCU ==
  g_u : Inport
  M_number : Inport  Port=2
  CVB_upper : MATLAB Function  TreatAsAtomicUnit=on
  g_unitaire_stack : Outport
  wires:
  g_u/1 -> CVB_upper/1(g)
  M_number/1 -> CVB_upper/2(M_number)
  CVB_upper/1(y) -> g_unitaire_stack/1

== system MMC_stack_centralized_HAAS_20260927/ /Sinus Modulation + Sorting Algorithm/M2 MCU ==
  g_u : Inport
  M_number : Inport  Port=2
  CVB_upper : MATLAB Function  TreatAsAtomicUnit=on
  g_unitaire_stack : Outport
  wires:
  g_u/1 -> CVB_upper/1(g)
  M_number/1 -> CVB_upper/2(M_number)
  CVB_upper/1(y) -> g_unitaire_stack/1

== system MMC_stack_centralized_HAAS_20260927/ /Sinus Modulation + Sorting Algorithm/M3 MCU ==
  g_u : Inport
  M_number : Inport  Port=2
  CVB_upper : MATLAB Function  TreatAsAtomicUnit=on
  g_unitaire_stack : Outport
  wires:
  g_u/1 -> CVB_upper/1(g)
  M_number/1 -> CVB_upper/2(M_number)
  CVB_upper/1(y) -> g_unitaire_stack/1

== system MMC_stack_centralized_HAAS_20260927/ /Sinus Modulation + Sorting Algorithm/M4 MCU ==
  g_u : Inport
  M_number : Inport  Port=2
  CVB_upper : MATLAB Function  TreatAsAtomicUnit=on
  g_unitaire_stack : Outport
  wires:
  g_u/1 -> CVB_upper/1(g)
  M_number/1 -> CVB_upper/2(M_number)
  CVB_upper/1(y) -> g_unitaire_stack/1

== system MMC_stack_centralized_HAAS_20260927/ /Sinus Modulation + Sorting Algorithm/M5 MCU ==
  g_u : Inport
  M_number : Inport  Port=2
  CVB_upper : MATLAB Function  TreatAsAtomicUnit=on
  g_unitaire_stack : Outport
  wires:
  g_u/1 -> CVB_upper/1(g)
  M_number/1 -> CVB_upper/2(M_number)
  CVB_upper/1(y) -> g_unitaire_stack/1

== system MMC_stack_centralized_HAAS_20260927/ /Sinus Modulation + Sorting Algorithm/Supervisor MCU ==
  note: NLM
  note: NLM
  note: Modulation reference
  note: Sorting and CVB algorithm - Upper and Lower stacks
  note: NLM modulation
  Vc_U : Inport
  I_U : Inport  Port=2
  Constant : Constant
  Constant1 : Constant  Value=0
  Constant4 : Constant  Value=a*1/2
  Gain : Gain  Gain=N
  Gain1 : Gain  Gain=m*1/2
  GreaterThan : RelationalOperator  Operator=~=  OutDataTypeStr=boolean  RndMeth=Simplest  InputSameDT=off
  Memory : Memory  InheritSampleTime=on  LinearizeMemory=on  LinearizeAsDelay=on
  Quantizer : Quantizer  QuantizationInterval=1
  Saturation : Saturate  UpperLimit=N  LowerLimit=0
  Sine Wave : Sin  Frequency=2*pi*f0  SampleTime=Ts
  Sorting_CVB_Upper : Subsystem
      settings: PortSchema="{\"entries\":[{\"content\":{\"sides\":[{\"content\":{\"connectorIds\":[\"In1\",\"In2\",\"In3\"]},\"type\":\"ConnectorPlacement.EquallySpacedRectSide\",\"uuid\":\"25566ff9-210a-4488-8b15-702d65e93a4b\"},{\"content\":{\"connectorIds\":[\"Out1\"],\"side\":\"RIGHT\"},\"type\":\"ConnectorPlacement.EquallySpacedRectSide\",\"uuid\":\"97373fc2-3782-4e65-8804-644d53fa5380\"},{\"content\":{\"connectorIds\":[\"In4\"],\"side\":\"TOP\"},\"type\":\"ConnectorPlacement.EquallySpacedRectSide\",\"uuid\":\"e65d2433-d029-4e4a-b081-22e9ded4f272\"}]},\"type\":\"ConnectorPlacement.EquallySpacedConnector\",\"uuid\":\"235c80e7-78ad-4e69-a231-ec76d675b4ae\"}],\"packageUris\":[\"http://schema.mathworks.com/mf0/Connector/R2020b\"],\"version\":\"1.0\"}"
  Sum1 : Sum  Inputs=|+-
  Switch : Switch  Criteria=u2 > Threshold  SaturateOnIntegerOverflow=off  InputSameDT=off
  gU : Outport
  tag scope: N_u=global, mu=global
  wires:
  Switch/1 -> Sorting_CVB_Upper/4(Pulse)
  Vc_U/1 -> Sorting_CVB_Upper/1(Vc_unitaire_stack)
  I_U/1 -> Sorting_CVB_Upper/2(i_stack)
  Sorting_CVB_Upper/1(g_unitaire_stack) -> gU/1
  Constant/1 -> Switch/1
  Sine Wave/1 -> Gain1/1
  Saturation/1 -> Sorting_CVB_Upper/3(N_on_stack), Memory/1, GreaterThan/1, [N_u]
  Constant1/1 -> Switch/3
  Quantizer/1 -> Saturation/1
  Gain/1 -> Quantizer/1
  GreaterThan/1 -> Switch/2
  Sum1/1 -> Gain/1, [mu]
  Gain1/1 -> Sum1/2
  Constant4/1 -> Sum1/1
  Memory/1 -> GreaterThan/2

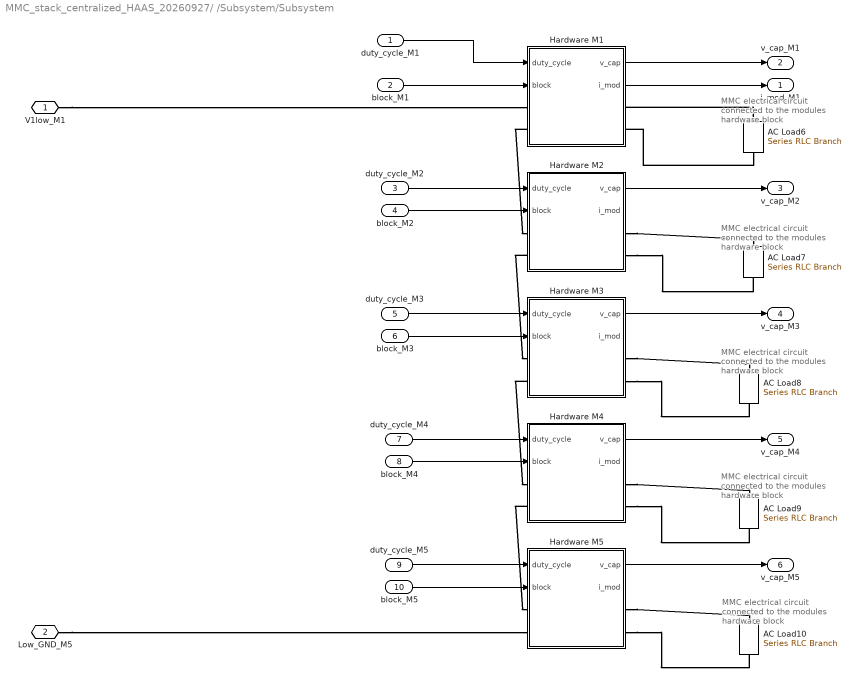
== system MMC_stack_centralized_HAAS_20260927/ /Subsystem/Subsystem ==
  note: MMC electrical circuit connected to the modules hardware block
  note: MMC electrical circuit connected to the modules hardware block
  note: MMC electrical circuit connected to the modules hardware block
  note: MMC electrical circuit connected to the modules hardware block
  note: MMC electrical circuit connected to the modules hardware block
  duty_cycle_M1 : Inport
  block_M1 : Inport  Port=2
  duty_cycle_M2 : Inport  Port=3
  block_M2 : Inport  Port=4
  duty_cycle_M3 : Inport  Port=5
  block_M3 : Inport  Port=6
  duty_cycle_M4 : Inport  Port=7
  block_M4 : Inport  Port=8
  duty_cycle_M5 : Inport  Port=9
  block_M5 : Inport  Port=10
  AC Load{6..10} (5 alike) : spsSeriesRLCBranchLib/Series RLC Branch  LConnTagsString=__new0  RConnTagsString=__new0  BranchType=C  Resistance=R  Inductance=L_arm  SetiL0=off  InitialCurrent=0  Capacitance=C_M_extra  Setx0=on  InitialVoltage=source_V  Measurements=None
  Hardware M1 : Subsystem
  Hardware M2 : Subsystem
  Hardware M3 : Subsystem
  Hardware M4 : Subsystem
  Hardware M5 : Subsystem
  V1low_M1 : PMIOPort  Side=Left
  Low_GND_M5 : PMIOPort  Port=2  Side=Left
  i_mod_M1 : Outport
  v_cap_M1 : Outport  Port=2
  v_cap_M2 : Outport  Port=3
  v_cap_M3 : Outport  Port=4
  v_cap_M4 : Outport  Port=5
  v_cap_M5 : Outport  Port=6
  wires:
  Hardware M1/1(v_cap) -> v_cap_M1/1
  duty_cycle_M1/1 -> Hardware M1/1(duty_cycle)
  duty_cycle_M2/1 -> Hardware M2/1(duty_cycle)
  block_M5/1 -> Hardware M5/2(block)
  Hardware M3/1(v_cap) -> v_cap_M3/1
  block_M1/1 -> Hardware M1/2(block)
  Hardware M1/2(i_mod) -> i_mod_M1/1
  duty_cycle_M4/1 -> Hardware M4/1(duty_cycle)
  block_M2/1 -> Hardware M2/2(block)
  Hardware M5/1(v_cap) -> v_cap_M5/1
  Hardware M2/1(v_cap) -> v_cap_M2/1
  duty_cycle_M3/1 -> Hardware M3/1(duty_cycle)
  duty_cycle_M5/1 -> Hardware M5/1(duty_cycle)
  block_M4/1 -> Hardware M4/2(block)
  block_M3/1 -> Hardware M3/2(block)
  Hardware M4/1(v_cap) -> v_cap_M4/1
  connections:
  Hardware M5/RConn2 -- AC Load10/RConn1
  AC Load6/LConn1 -- Hardware M1/RConn1
  Hardware M1/LConn2 -- Hardware M2/LConn1
  Hardware M3/LConn2 -- Hardware M4/LConn1
  Hardware M5/RConn1 -- AC Load10/LConn1
  AC Load6/RConn1 -- Hardware M1/RConn2
  Hardware M2/RConn2 -- AC Load7/RConn1
  Hardware M2/LConn2 -- Hardware M3/LConn1
  Hardware M2/RConn1 -- AC Load7/LConn1
  Hardware M3/RConn1 -- AC Load8/LConn1
  Hardware M3/RConn2 -- AC Load8/RConn1
  Hardware M4/RConn2 -- AC Load9/RConn1
  Hardware M4/RConn1 -- AC Load9/LConn1
  Hardware M4/LConn2 -- Hardware M5/LConn1
  V1low_M1/RConn1 -- Hardware M1/LConn1
  Low_GND_M5/RConn1 -- Hardware M5/LConn2

== system MMC_stack_centralized_HAAS_20260927/ /Communication_subsystem/Upper_arm/M1_Comm ==
  TX_variables : Inport
  sync : Inport  Port=2
  RX_signal : Inport  Port=3
  Data Type Conversion : DataTypeConversion  OutDataTypeStr=single  SaturateOnIntegerOverflow=off  RndMeth=Floor
  Delay : Delay  DelayLength=Tcom_sample
  Delay1 : Delay  DelayLength=1
  Delay2 : Delay  DelayLength=1
  Scope : Scope  NumInputPorts=6
  Scope1 : Scope  NumInputPorts=2
  Snapshot : MATLAB Function  TreatAsAtomicUnit=on
  TxFormatter : MATLAB Function  TreatAsAtomicUnit=on
  node_id : Constant
  TX_signal : Outport
  RX_Variables : Outport  Port=2
  wires:
  TX_variables/1 -> Data Type Conversion/1
  TxFormatter/1(tx_data) -> Delay/1
  Delay/1 -> TX_signal/1
  sync/1 -> Snapshot/3(sync), Scope1/1, TxFormatter/2(sync)  "Ctrl_task"
  RX_signal/1 -> Snapshot/1(rx_signal), TxFormatter/3(rx_signal)
  Snapshot/1(rx_variables) -> RX_Variables/1
  Data Type Conversion/1 -> TxFormatter/1(tx_variables)
  node_id/1 -> TxFormatter/4(node_id)
  TxFormatter/2(tx_fire) -> Scope/1
  TxFormatter/3(tx_busy) -> Scope/2
  TxFormatter/5(rx_count_dbg) -> Scope/4
  TxFormatter/6(rx_id_dbg) -> Scope1/2, Scope/5  "1 -> 2 data"
  TxFormatter/7(overrun) -> Scope/6
  TxFormatter/8(local_frame_snapshot) -> Delay1/1
  Delay1/1 -> Snapshot/2(local_frame_snapshot)
  TxFormatter/4(round_done) -> Scope/3, Delay2/1
  Delay2/1 -> Snapshot/4(round_done)

== system MMC_stack_centralized_HAAS_20260927/ /Communication_subsystem/Upper_arm/M2_Comm ==
  TX_variables : Inport
  sync : Inport  Port=2
  RX_signal : Inport  Port=3
  Data Type Conversion : DataTypeConversion  OutDataTypeStr=single  SaturateOnIntegerOverflow=off  RndMeth=Floor
  Delay : Delay  DelayLength=Tcom_sample
  Delay1 : Delay  DelayLength=1
  Scope : Scope  NumInputPorts=6
  Snapshot : MATLAB Function  TreatAsAtomicUnit=on
  TxFormatter : MATLAB Function  TreatAsAtomicUnit=on
  node_id : Constant  Value=2
  TX_signal : Outport
  RX_Variables : Outport  Port=2
  wires:
  TxFormatter/2(tx_fire) -> Scope/1
  TxFormatter/3(tx_busy) -> Scope/2
  TxFormatter/8(local_frame_snapshot) -> Delay1/1
  TxFormatter/7(overrun) -> Scope/6
  TX_variables/1 -> Data Type Conversion/1
  Delay/1 -> TX_signal/1
  TxFormatter/4(round_done) -> Scope/3
  Snapshot/1(rx_variables) -> RX_Variables/1
  TxFormatter/1(tx_data) -> Delay/1
  Delay1/1 -> Snapshot/2(local_frame_snapshot)
  Data Type Conversion/1 -> TxFormatter/1(tx_variables)
  sync/1 -> Snapshot/3(sync), TxFormatter/2(sync)
  node_id/1 -> TxFormatter/4(node_id)
  TxFormatter/6(rx_id_dbg) -> Scope/5
  RX_signal/1 -> Snapshot/1(rx_signal), TxFormatter/3(rx_signal)
  TxFormatter/5(rx_count_dbg) -> Scope/4

== system MMC_stack_centralized_HAAS_20260927/ /Communication_subsystem/Upper_arm/M3_Comm ==
  TX_variables : Inport
  sync : Inport  Port=2
  RX_signal : Inport  Port=3
  Data Type Conversion : DataTypeConversion  OutDataTypeStr=single  SaturateOnIntegerOverflow=off  RndMeth=Floor
  Delay : Delay  DelayLength=Tcom_sample
  Delay1 : Delay  DelayLength=1
  Scope : Scope  NumInputPorts=6
  Snapshot : MATLAB Function  TreatAsAtomicUnit=on
  TxFormatter : MATLAB Function  TreatAsAtomicUnit=on
  node_id : Constant  Value=3
  TX_signal : Outport
  RX_Variables : Outport  Port=2
  wires:
  TxFormatter/2(tx_fire) -> Scope/1
  TxFormatter/3(tx_busy) -> Scope/2
  TxFormatter/8(local_frame_snapshot) -> Delay1/1
  TxFormatter/7(overrun) -> Scope/6
  TX_variables/1 -> Data Type Conversion/1
  Delay/1 -> TX_signal/1
  TxFormatter/4(round_done) -> Scope/3
  Snapshot/1(rx_variables) -> RX_Variables/1
  TxFormatter/1(tx_data) -> Delay/1
  Delay1/1 -> Snapshot/2(local_frame_snapshot)
  Data Type Conversion/1 -> TxFormatter/1(tx_variables)
  sync/1 -> Snapshot/3(sync), TxFormatter/2(sync)
  node_id/1 -> TxFormatter/4(node_id)
  TxFormatter/6(rx_id_dbg) -> Scope/5
  RX_signal/1 -> Snapshot/1(rx_signal), TxFormatter/3(rx_signal)
  TxFormatter/5(rx_count_dbg) -> Scope/4

== system MMC_stack_centralized_HAAS_20260927/ /Communication_subsystem/Upper_arm/M4_Comm ==
  TX_variables : Inport
  sync : Inport  Port=2
  RX_signal : Inport  Port=3
  Data Type Conversion : DataTypeConversion  OutDataTypeStr=single  SaturateOnIntegerOverflow=off  RndMeth=Floor
  Delay : Delay  DelayLength=Tcom_sample
  Delay1 : Delay  DelayLength=1
  Scope : Scope  NumInputPorts=6
  Snapshot : MATLAB Function  TreatAsAtomicUnit=on
  TxFormatter : MATLAB Function  TreatAsAtomicUnit=on
  node_id : Constant  Value=4
  TX_signal : Outport
  RX_Variables : Outport  Port=2
  wires:
  TxFormatter/2(tx_fire) -> Scope/1
  TxFormatter/3(tx_busy) -> Scope/2
  TxFormatter/8(local_frame_snapshot) -> Delay1/1
  TxFormatter/7(overrun) -> Scope/6
  TX_variables/1 -> Data Type Conversion/1
  Delay/1 -> TX_signal/1
  TxFormatter/4(round_done) -> Scope/3
  Snapshot/1(rx_variables) -> RX_Variables/1
  TxFormatter/1(tx_data) -> Delay/1
  Delay1/1 -> Snapshot/2(local_frame_snapshot)
  Data Type Conversion/1 -> TxFormatter/1(tx_variables)
  sync/1 -> Snapshot/3(sync), TxFormatter/2(sync)
  node_id/1 -> TxFormatter/4(node_id)
  TxFormatter/6(rx_id_dbg) -> Scope/5
  RX_signal/1 -> Snapshot/1(rx_signal), TxFormatter/3(rx_signal)
  TxFormatter/5(rx_count_dbg) -> Scope/4

== system MMC_stack_centralized_HAAS_20260927/ /Communication_subsystem/Upper_arm/M5_Comm ==
  TX_variables : Inport
  sync : Inport  Port=2
  RX_signal : Inport  Port=3
  Data Type Conversion : DataTypeConversion  OutDataTypeStr=single  SaturateOnIntegerOverflow=off  RndMeth=Floor
  Delay : Delay  DelayLength=Tcom_sample
  Delay1 : Delay  DelayLength=1
  Scope : Scope  NumInputPorts=6
  Snapshot : MATLAB Function  TreatAsAtomicUnit=on
  TxFormatter : MATLAB Function  TreatAsAtomicUnit=on
  node_id : Constant  Value=5
  TX_signal : Outport
  RX_Variables : Outport  Port=2
  wires:
  TxFormatter/2(tx_fire) -> Scope/1
  TxFormatter/3(tx_busy) -> Scope/2
  TxFormatter/8(local_frame_snapshot) -> Delay1/1
  TxFormatter/7(overrun) -> Scope/6
  TX_variables/1 -> Data Type Conversion/1
  Delay/1 -> TX_signal/1
  TxFormatter/4(round_done) -> Scope/3
  Snapshot/1(rx_variables) -> RX_Variables/1
  TxFormatter/1(tx_data) -> Delay/1
  Delay1/1 -> Snapshot/2(local_frame_snapshot)
  Data Type Conversion/1 -> TxFormatter/1(tx_variables)
  sync/1 -> Snapshot/3(sync), TxFormatter/2(sync)
  node_id/1 -> TxFormatter/4(node_id)
  TxFormatter/6(rx_id_dbg) -> Scope/5
  RX_signal/1 -> Snapshot/1(rx_signal), TxFormatter/3(rx_signal)
  TxFormatter/5(rx_count_dbg) -> Scope/4

== system MMC_stack_centralized_HAAS_20260927/ /Sinus Modulation + Sorting Algorithm/Supervisor MCU/Sorting_CVB_Upper ==
  Vc_unitaire_stack : Inport
  i_stack : Inport  Port=2
  N_on_stack : Inport  Port=3
  Pulse : Inport  Port=4
  CVB : MATLAB Function  TreatAsAtomicUnit=on
  Constant : Constant  Value=duty_cycle
  Scope : Scope  NumInputPorts=5
  Sorting : Subsystem
  g_unitaire_stack : Outport
  wires:
  Vc_unitaire_stack/1 -> Sorting/1(Vc_u), Scope/1
  Sorting/1(Ordre_u) -> CVB/1(ordre)
  N_on_stack/1 -> Scope/4, CVB/3(N_on)
  i_stack/1 -> Scope/2, Sorting/2(i_u)
  Sorting/2(Sens_u) -> CVB/2(sens)
  Pulse/1 -> Scope/5, Sorting/Enable
  CVB/1(y) -> Scope/3, g_unitaire_stack/1
  Constant/1 -> CVB/4(duty_cycle)
